simulink model "soft_robot_model"  (R2025b)
settings: Solver=VariableStepAuto  StartTime=0.0  StopTime=10.0  RelTol=1e-3
values from neighbouring files (symbols this model uses):
  d_z = 0    [Code4Simulink.m]
  L = 0.15    [Code4Simulink.m]
  phi = [30, 150, 270] * pi/180    [Code4Simulink.m]
  theta_x = deg2rad(0)    [Code4Simulink.m]
  theta_y = deg2rad(0)    [Code4Simulink.m]
undefined symbols (not defined in the file or in its folder): X, Y, Z
libraries: sm_lib x23, nesl_utility x4
settings Model: Creator=didar  LastModifiedBy=didar

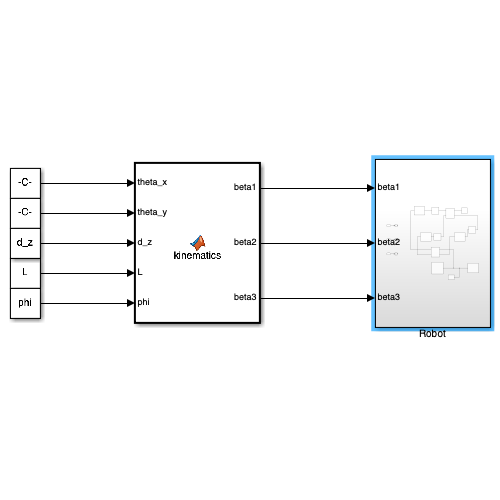
[thumbnail: Simulink's stored preview of the top-level diagram]
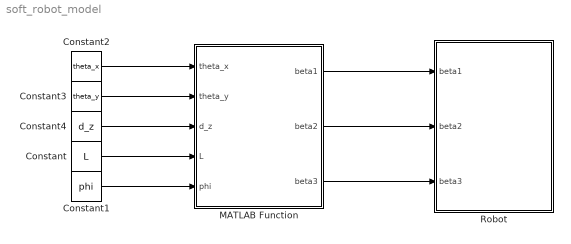
== system soft_robot_model ==
  Constant : Constant  Value=L
  Constant1 : Constant  Value=phi
  Constant2 : Constant  Value=theta_x
  Constant3 : Constant  Value=theta_y
  Constant4 : Constant  Value=d_z
  MATLAB Function : MATLAB Function  TreatAsAtomicUnit=on
  Robot : Subsystem
  wires:
  Constant1/1 -> MATLAB Function/5(phi)
  Constant/1 -> MATLAB Function/4(L)
  Constant2/1 -> MATLAB Function/1(theta_x)
  Constant3/1 -> MATLAB Function/2(theta_y)
  Constant4/1 -> MATLAB Function/3(d_z)
  MATLAB Function/1(beta1) -> Robot/1(beta1)
  MATLAB Function/2(beta2) -> Robot/2(beta2)
  MATLAB Function/3(beta3) -> Robot/3(beta3)

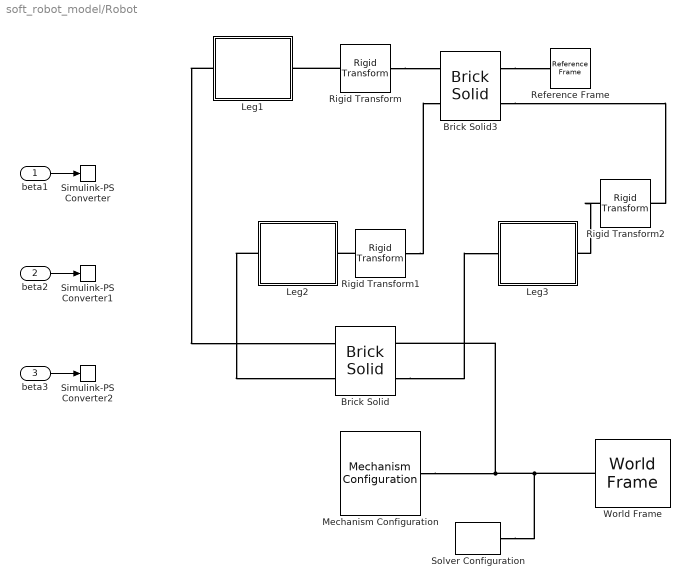
== system soft_robot_model/Robot ==
  beta1 : Inport
  beta2 : Inport  Port=2
  beta3 : Inport  Port=3
  Brick Solid : sm_lib/Body Elements/Brick Solid  BrickDimensions=[10 10 1]  BrickDimensionsUnits=cm  ExportEntireGeometry=off  InertiaType=CalculateFromGeometry  BasedOnType=Density  Density=1000  DensityUnits=kg/m^3  Mass=1  MassUnits=kg  CenterOfMass=[0 0 0]  CenterOfMassUnits=m  MomentsOfInertia=[1 1 1]  MomentsOfInertiaUnits=kg*m^2  ProductsOfInertia=[0 0 0]  ProductsOfInertiaUnits=kg*m^2  GraphicType=FromGeometry  MarkerShape=Sphere  MarkerSize=10  GraphicVisPropType=SimpleVisualProperties  GraphicDiffuseColor=[0.5 0.5 0.5]  GraphicOpacity=1  GraphicSpecularColor=[0.5 0.5 0.5 1.0]  GraphicAmbientColor=[0.15 0.15 0.15 1.0]  GraphicEmissiveColor=[0.0 0.0 0.0 1.0]  GraphicShininess=75  DoExposeReferenceFrame=on  SerializedFrames=<Frames><Frame><Id>Frame1</Id><Value><Name>F1</Name><Origin><Source>ReferenceFrame</Source><FeatureName></FeatureName></Origin><PrimaryAxis><DefinedDirection>+Z</DefinedDirection><Source>ReferenceFrame</Source><SourceDirection>+Z</SourceDirection><FeatureName></FeatureName></PrimaryAxis><SecondaryAxis><DefinedDirection>+X</DefinedDirection><Source>ReferenceFrame</Source><SourceDirection>+X</SourceDirection><FeatureName></FeatureName></SecondaryAxis></Value></Frame><Frame><Id>Frame2</Id><Value><Name>F2</Name><Origin><Source>ReferenceFrame</Source><FeatureName></FeatureName></Origin><PrimaryAxis><DefinedDirection>+Z</DefinedDirection><Source>ReferenceFrame</Source><SourceDirection>+Z</SourceDirection><FeatureName></FeatureName></PrimaryAxis><SecondaryAxis><DefinedDirection>+X</DefinedDirection><Source>ReferenceFrame</Source><SourceDirection>+X</SourceDirection><FeatureName></FeatureName></SecondaryAxis></Value></Frame><Frame><Id>Frame3</Id><Value><Name>F3</Name><Origin><Source>ReferenceFrame</Source><FeatureName></FeatureName></Origin><PrimaryAxis><DefinedDirection>+Z</DefinedDirection><Source>ReferenceFrame</Source><SourceDirection>+Z</SourceDirection><FeatureName></FeatureName></PrimaryAxis><SecondaryAxis><DefinedDirection>+X</DefinedDirection><Source>ReferenceFrame</Source><SourceDirection>+X</SourceDirection><FeatureName></FeatureName></SecondaryAxis></Value></Frame></Frames>
  Brick Solid3 : sm_lib/Body Elements/Brick Solid  BrickDimensions=[10 10 1]  BrickDimensionsUnits=cm  ExportEntireGeometry=off  InertiaType=CalculateFromGeometry  BasedOnType=Density  Density=1000  DensityUnits=kg/m^3  Mass=1  MassUnits=kg  CenterOfMass=[0 0 0]  CenterOfMassUnits=m  MomentsOfInertia=[1 1 1]  MomentsOfInertiaUnits=kg*m^2  ProductsOfInertia=[0 0 0]  ProductsOfInertiaUnits=kg*m^2  GraphicType=FromGeometry  MarkerShape=Sphere  MarkerSize=10  GraphicVisPropType=SimpleVisualProperties  GraphicDiffuseColor=[0.5 0.5 0.5]  GraphicOpacity=1  GraphicSpecularColor=[0.5 0.5 0.5 1.0]  GraphicAmbientColor=[0.15 0.15 0.15 1.0]  GraphicEmissiveColor=[0.0 0.0 0.0 1.0]  GraphicShininess=75  DoExposeReferenceFrame=on  SerializedFrames=<Frames><Frame><Id>Frame1</Id><Value><Name>F1</Name><Origin><Source>ReferenceFrame</Source><FeatureName></FeatureName></Origin><PrimaryAxis><DefinedDirection>+Z</DefinedDirection><Source>ReferenceFrame</Source><SourceDirection>+Z</SourceDirection><FeatureName></FeatureName></PrimaryAxis><SecondaryAxis><DefinedDirection>+X</DefinedDirection><Source>ReferenceFrame</Source><SourceDirection>+X</SourceDirection><FeatureName></FeatureName></SecondaryAxis></Value></Frame><Frame><Id>Frame2</Id><Value><Name>F2</Name><Origin><Source>ReferenceFrame</Source><FeatureName></FeatureName></Origin><PrimaryAxis><DefinedDirection>+Z</DefinedDirection><Source>ReferenceFrame</Source><SourceDirection>+Z</SourceDirection><FeatureName></FeatureName></PrimaryAxis><SecondaryAxis><DefinedDirection>+X</DefinedDirection><Source>ReferenceFrame</Source><SourceDirection>+X</SourceDirection><FeatureName></FeatureName></SecondaryAxis></Value></Frame><Frame><Id>Frame3</Id><Value><Name>F3</Name><Origin><Source>ReferenceFrame</Source><FeatureName></FeatureName></Origin><PrimaryAxis><DefinedDirection>+Z</DefinedDirection><Source>ReferenceFrame</Source><SourceDirection>+Z</SourceDirection><FeatureName></FeatureName></PrimaryAxis><SecondaryAxis><DefinedDirection>+X</DefinedDirection><Source>ReferenceFrame</Source><SourceDirection>+X</SourceDirection><FeatureName></FeatureName></SecondaryAxis></Value></Frame></Frames>
  Leg1 : Subsystem
  Leg2 : Subsystem
  Leg3 : Subsystem
  Mechanism Configuration : sm_lib/Utilities/Mechanism Configuration  UniformGravity=Constant  GravityVector=[0 0 -9.80665]  GravityVectorUnits=m/s^2  LinearizationDelta=0.001  JointModeTransitionNonlinearIterations=2
  Reference Frame : sm_lib/Frames and Transforms/Reference Frame
  Rigid Transform : sm_lib/Frames and Transforms/Rigid Transform  RotationMethod=StandardAxis  FollAlignAxisA=+X  BaseAlignAxisA=+Y  FollAlignAxisB=+Y  BaseAlignAxisB=+Z  RotationStandardAxis=+Z  RotationAngle=30  RotationAngleUnits=deg  RotationArbitraryAxis=[0 0 1]  RotationSequenceAxes=FollowerAxes  RotationSequence=XYX  RotationSequenceAngles=[0 0 0]  RotationSequenceAnglesUnits=deg  RotationMatrix=[1 0 0;0 1 0;0 0 1]  Quaternion=[1 0 0 0]  TranslationMethod=None  TranslationCartesianOffset=[0 0 0]  TranslationCartesianOffsetUnits=m  TranslationStandardAxis=+Z  TranslationStandardOffset=0  TranslationStandardOffsetUnits=m  TranslationROffset=0  TranslationROffsetUnits=m  TranslationThetaOffset=0  TranslationThetaOffsetUnits=deg  TranslationZOffset=0  TranslationZOffsetUnits=m
  Rigid Transform1 : sm_lib/Frames and Transforms/Rigid Transform  RotationMethod=StandardAxis  FollAlignAxisA=+X  BaseAlignAxisA=+Y  FollAlignAxisB=+Y  BaseAlignAxisB=+Z  RotationStandardAxis=+Z  RotationAngle=150  RotationAngleUnits=deg  RotationArbitraryAxis=[0 0 1]  RotationSequenceAxes=FollowerAxes  RotationSequence=XYX  RotationSequenceAngles=[0 0 0]  RotationSequenceAnglesUnits=deg  RotationMatrix=[1 0 0;0 1 0;0 0 1]  Quaternion=[1 0 0 0]  TranslationMethod=None  TranslationCartesianOffset=[0 0 0]  TranslationCartesianOffsetUnits=m  TranslationStandardAxis=+Z  TranslationStandardOffset=0  TranslationStandardOffsetUnits=m  TranslationROffset=0  TranslationROffsetUnits=m  TranslationThetaOffset=0  TranslationThetaOffsetUnits=deg  TranslationZOffset=0  TranslationZOffsetUnits=m
  Rigid Transform2 : sm_lib/Frames and Transforms/Rigid Transform  RotationMethod=StandardAxis  FollAlignAxisA=+X  BaseAlignAxisA=+Y  FollAlignAxisB=+Y  BaseAlignAxisB=+Z  RotationStandardAxis=+Z  RotationAngle=270  RotationAngleUnits=deg  RotationArbitraryAxis=[0 0 1]  RotationSequenceAxes=FollowerAxes  RotationSequence=XYX  RotationSequenceAngles=[0 0 0]  RotationSequenceAnglesUnits=deg  RotationMatrix=[1 0 0;0 1 0;0 0 1]  Quaternion=[1 0 0 0]  TranslationMethod=None  TranslationCartesianOffset=[0 0 0]  TranslationCartesianOffsetUnits=m  TranslationStandardAxis=+Z  TranslationStandardOffset=0  TranslationStandardOffsetUnits=m  TranslationROffset=0  TranslationROffsetUnits=m  TranslationThetaOffset=0  TranslationThetaOffsetUnits=deg  TranslationZOffset=0  TranslationZOffsetUnits=m
  Simulink-PS Converter : nesl_utility/Simulink-PS Converter  PhysicalDomain=network_engine_domain  SubClassName=ps_input  LeftPortType=input  RightPortType=output  PseudoPeriodic=off  Frequencies=[]  NoiseDistribution=none  NoiseParameters=[]  Unit=1  AffineConversion=off  FilteringAndDerivatives=provide  SimscapeFilterOrder=1  InputFilterTimeConstant=0.001  UdotUserProvided=0
  Simulink-PS Converter1 : nesl_utility/Simulink-PS Converter  PhysicalDomain=network_engine_domain  SubClassName=ps_input  LeftPortType=input  RightPortType=output  PseudoPeriodic=off  Frequencies=[]  NoiseDistribution=none  NoiseParameters=[]  Unit=1  AffineConversion=off  FilteringAndDerivatives=provide  SimscapeFilterOrder=1  InputFilterTimeConstant=0.001  UdotUserProvided=0
  Simulink-PS Converter2 : nesl_utility/Simulink-PS Converter  PhysicalDomain=network_engine_domain  SubClassName=ps_input  LeftPortType=input  RightPortType=output  PseudoPeriodic=off  Frequencies=[]  NoiseDistribution=none  NoiseParameters=[]  Unit=1  AffineConversion=off  FilteringAndDerivatives=provide  SimscapeFilterOrder=1  InputFilterTimeConstant=0.001  UdotUserProvided=0
  Solver Configuration : nesl_utility/Solver Configuration  PhysicalDomain=network_engine_domain  SubClassName=solver  LeftPortType=input  RightPortType=generic  Tones=[]  Harmonics=[]  SimulateNoise=off  Profile=off  UseLocalSampling=off  EnableSwitchedLinearOptims=on  FrequencyDomain=off  UseCCode=off  RelTol=0.001  AbsTol=0.001  MinStep=1e-09  ToWorkspace=off  RevertToSquareIcSolve=off  NumHomotopyIterations=100  PhasorMode=off  PhasorModeNumHarmonics=1  ConsistencySolver=NEWTON_XTOL_AFTER_FTOL  IndexReductionMethod=DerivativeReplacement  DoDC=off  ResidualTolerance=1e-09  ConsistencyTolSource=GLOBAL  ConsistencyAbsTol=0.001  ConsistencyRelTol=0.001  ConsistencyTolFactor=0.001  UseLocalSolver=off  LocalSolverChoice=NE_BACKWARD_EULER_ADVANCER  ResolveIndetEquations=on  FunctionEvalNumThread=1  LocalSolverSampleTime=0.001  DoFixedCost=off  MaxNonlinIter=3  MaxModeIter=2  ComputeImpulses=off  ImpulseIterations=2  LinearAlgebra=auto  LinearAlgebraNumThread=0  EquationFormulation=NE_TIME_EF  DelaysMemoryBudget=1024  AutomaticFiltering=on  FilteringTimeConstant=0.001  PartitionStorageMethod=AS_NEEDED  PartitionMemoryBudget=1024  PartitionMethod=ROBUST  MultibodyUseLocalSolver=off  MultibodyLocalSolverChoice=ODE1  MultibodyLocalSolverSampleTime=0.001
  World Frame : sm_lib/Frames and Transforms/World Frame
  wires:
  beta1/1 -> Simulink-PS Converter/1
  beta2/1 -> Simulink-PS Converter1/1
  beta3/1 -> Simulink-PS Converter2/1
  connections:
  World Frame/RConn1 -- Solver Configuration/RConn1 -- Brick Solid/RConn1 -- Mechanism Configuration/RConn1
  Leg1/RConn1 -- Brick Solid/LConn1
  Leg2/RConn1 -- Brick Solid/LConn2
  Brick Solid/RConn2 -- Leg3/RConn1
  Rigid Transform/LConn1 -- Leg1/LConn1
  Rigid Transform/RConn1 -- Brick Solid3/LConn1
  Rigid Transform1/LConn1 -- Leg2/LConn1
  Rigid Transform1/RConn1 -- Brick Solid3/LConn2
  Rigid Transform2/LConn1 -- Leg3/LConn1
  Brick Solid3/RConn2 -- Rigid Transform2/RConn1
  Brick Solid3/RConn1 -- Reference Frame/RConn1

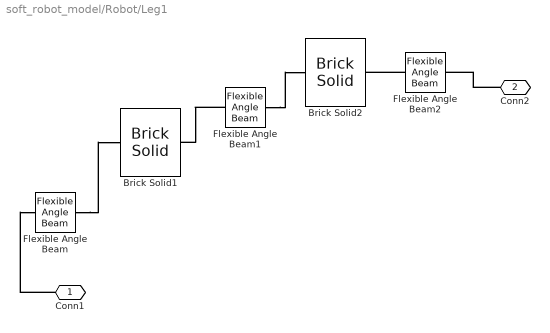
== system soft_robot_model/Robot/Leg1 ==
  Brick Solid1 : sm_lib/Body Elements/Brick Solid  BrickDimensions=[4.5 0.7 8.6]  BrickDimensionsUnits=cm  ExportEntireGeometry=off  InertiaType=CalculateFromGeometry  BasedOnType=Density  Density=1000  DensityUnits=kg/m^3  Mass=1  MassUnits=kg  CenterOfMass=[0 0 0]  CenterOfMassUnits=m  MomentsOfInertia=[1 1 1]  MomentsOfInertiaUnits=kg*m^2  ProductsOfInertia=[0 0 0]  ProductsOfInertiaUnits=kg*m^2  GraphicType=FromGeometry  MarkerShape=Sphere  MarkerSize=10  GraphicVisPropType=SimpleVisualProperties  GraphicDiffuseColor=[0.5 0.5 0.5]  GraphicOpacity=1  GraphicSpecularColor=[0.5 0.5 0.5 1.0]  GraphicAmbientColor=[0.15 0.15 0.15 1.0]  GraphicEmissiveColor=[0.0 0.0 0.0 1.0]  GraphicShininess=75  DoExposeReferenceFrame=on  SerializedFrames=<Frames><Frame><Id>Frame1</Id><Value><Name>F1</Name><Origin><Source>ReferenceFrame</Source><FeatureName></FeatureName></Origin><PrimaryAxis><DefinedDirection>+Z</DefinedDirection><Source>ReferenceFrame</Source><SourceDirection>+Z</SourceDirection><FeatureName></FeatureName></PrimaryAxis><SecondaryAxis><DefinedDirection>+X</DefinedDirection><Source>ReferenceFrame</Source><SourceDirection>+X</SourceDirection><FeatureName></FeatureName></SecondaryAxis></Value></Frame></Frames>
  Brick Solid2 : sm_lib/Body Elements/Brick Solid  BrickDimensions=[4.5 0.7 8.6]  BrickDimensionsUnits=cm  ExportEntireGeometry=off  InertiaType=CalculateFromGeometry  BasedOnType=Density  Density=1000  DensityUnits=kg/m^3  Mass=1  MassUnits=kg  CenterOfMass=[0 0 0]  CenterOfMassUnits=m  MomentsOfInertia=[1 1 1]  MomentsOfInertiaUnits=kg*m^2  ProductsOfInertia=[0 0 0]  ProductsOfInertiaUnits=kg*m^2  GraphicType=FromGeometry  MarkerShape=Sphere  MarkerSize=10  GraphicVisPropType=SimpleVisualProperties  GraphicDiffuseColor=[0.5 0.5 0.5]  GraphicOpacity=1  GraphicSpecularColor=[0.5 0.5 0.5 1.0]  GraphicAmbientColor=[0.15 0.15 0.15 1.0]  GraphicEmissiveColor=[0.0 0.0 0.0 1.0]  GraphicShininess=75  DoExposeReferenceFrame=on  SerializedFrames=<Frames><Frame><Id>Frame1</Id><Value><Name>F1</Name><Origin><Source>ReferenceFrame</Source><FeatureName></FeatureName></Origin><PrimaryAxis><DefinedDirection>+Z</DefinedDirection><Source>ReferenceFrame</Source><SourceDirection>+Z</SourceDirection><FeatureName></FeatureName></PrimaryAxis><SecondaryAxis><DefinedDirection>+X</DefinedDirection><Source>ReferenceFrame</Source><SourceDirection>+X</SourceDirection><FeatureName></FeatureName></SecondaryAxis></Value></Frame></Frames>
  Flexible Angle Beam : sm_lib/Body Elements/Flexible Bodies/Beams/Flexible Angle Beam  EndToEndWidth=1  EndToEndWidthUnits=m  EndToEndHeight=1  EndToEndHeightUnits=m  VerticalLegThickness=0.1  VerticalLegThicknessUnits=m  HorizontalLegThickness=0.1  HorizontalLegThicknessUnits=m  Length=10  LengthUnits=m  StiffnessAndInertiaType=CalculateFromGeometry  Density=2700  DensityUnits=kg/m^3  ModuliType=YoungsPoissons  YoungsModulus=70  YoungsModulusUnits=GPa  PoissonsRatio=0.33  ShearModulus=26  ShearModulusUnits=GPa  GeometricCentroid=[0 0]  GeometricCentroidUnits=m  BendingCentroid=[0 0]  BendingCentroidUnits=m  ShearCenter=[0 0]  ShearCenterUnits=m  AxialRigidity=1  AxialRigidityUnits=Pa*m^2  FlexuralRigidity=[1 1]  FlexuralRigidityUnits=Pa*m^4  CrossFlexuralRigidity=0  CrossFlexuralRigidityUnits=Pa*m^4  TorsionalRigidity=1  TorsionalRigidityUnits=Pa*m^4  CenterOfMass=[0 0]  CenterOfMassUnits=m  MassPerUnitLength=1  MassPerUnitLengthUnits=kg/m  MassMomentOfInertiaDensity=[1 1]  MassMomentOfInertiaDensityUnits=kg*m  MassProductOfInertiaDensity=0  MassProductOfInertiaDensityUnits=kg*m  DampingType=Proportional  ProportionalDampingAlpha=0  ProportionalDampingAlphaUnits=1/s  ProportionalDampingBeta=0.001  ProportionalDampingBetaUnits=s  UniformModalDampingRatio=0.01  NumElements=1  ReferenceConditionsType=LinearizedMeanAxes  DoExposeReferenceFrame=off  ReductionType=None  NumRetainedModes=1  GraphicType=FromGeometry  GraphicVisPropType=SimpleVisualProperties  GraphicDiffuseColor=[0.5 0.5 0.5]  GraphicOpacity=1  GraphicSpecularColor=[0.5 0.5 0.5 1.0]  GraphicAmbientColor=[0.15 0.15 0.15 1.0]  GraphicEmissiveColor=[0.0 0.0 0.0 1.0]  GraphicShininess=75  DoExposeZminFrame=on  DoExposeZmaxFrame=on  SerializedFrames=<Frames/>
  Flexible Angle Beam1 : sm_lib/Body Elements/Flexible Bodies/Beams/Flexible Angle Beam  EndToEndWidth=1  EndToEndWidthUnits=m  EndToEndHeight=1  EndToEndHeightUnits=m  VerticalLegThickness=0.1  VerticalLegThicknessUnits=m  HorizontalLegThickness=0.1  HorizontalLegThicknessUnits=m  Length=10  LengthUnits=m  StiffnessAndInertiaType=CalculateFromGeometry  Density=2700  DensityUnits=kg/m^3  ModuliType=YoungsPoissons  YoungsModulus=70  YoungsModulusUnits=GPa  PoissonsRatio=0.33  ShearModulus=26  ShearModulusUnits=GPa  GeometricCentroid=[0 0]  GeometricCentroidUnits=m  BendingCentroid=[0 0]  BendingCentroidUnits=m  ShearCenter=[0 0]  ShearCenterUnits=m  AxialRigidity=1  AxialRigidityUnits=Pa*m^2  FlexuralRigidity=[1 1]  FlexuralRigidityUnits=Pa*m^4  CrossFlexuralRigidity=0  CrossFlexuralRigidityUnits=Pa*m^4  TorsionalRigidity=1  TorsionalRigidityUnits=Pa*m^4  CenterOfMass=[0 0]  CenterOfMassUnits=m  MassPerUnitLength=1  MassPerUnitLengthUnits=kg/m  MassMomentOfInertiaDensity=[1 1]  MassMomentOfInertiaDensityUnits=kg*m  MassProductOfInertiaDensity=0  MassProductOfInertiaDensityUnits=kg*m  DampingType=Proportional  ProportionalDampingAlpha=0  ProportionalDampingAlphaUnits=1/s  ProportionalDampingBeta=0.001  ProportionalDampingBetaUnits=s  UniformModalDampingRatio=0.01  NumElements=1  ReferenceConditionsType=LinearizedMeanAxes  DoExposeReferenceFrame=off  ReductionType=None  NumRetainedModes=1  GraphicType=FromGeometry  GraphicVisPropType=SimpleVisualProperties  GraphicDiffuseColor=[0.5 0.5 0.5]  GraphicOpacity=1  GraphicSpecularColor=[0.5 0.5 0.5 1.0]  GraphicAmbientColor=[0.15 0.15 0.15 1.0]  GraphicEmissiveColor=[0.0 0.0 0.0 1.0]  GraphicShininess=75  DoExposeZminFrame=on  DoExposeZmaxFrame=on  SerializedFrames=<Frames/>
  Flexible Angle Beam2 : sm_lib/Body Elements/Flexible Bodies/Beams/Flexible Angle Beam  EndToEndWidth=1  EndToEndWidthUnits=m  EndToEndHeight=1  EndToEndHeightUnits=m  VerticalLegThickness=0.1  VerticalLegThicknessUnits=m  HorizontalLegThickness=0.1  HorizontalLegThicknessUnits=m  Length=10  LengthUnits=m  StiffnessAndInertiaType=CalculateFromGeometry  Density=2700  DensityUnits=kg/m^3  ModuliType=YoungsPoissons  YoungsModulus=70  YoungsModulusUnits=GPa  PoissonsRatio=0.33  ShearModulus=26  ShearModulusUnits=GPa  GeometricCentroid=[0 0]  GeometricCentroidUnits=m  BendingCentroid=[0 0]  BendingCentroidUnits=m  ShearCenter=[0 0]  ShearCenterUnits=m  AxialRigidity=1  AxialRigidityUnits=Pa*m^2  FlexuralRigidity=[1 1]  FlexuralRigidityUnits=Pa*m^4  CrossFlexuralRigidity=0  CrossFlexuralRigidityUnits=Pa*m^4  TorsionalRigidity=1  TorsionalRigidityUnits=Pa*m^4  CenterOfMass=[0 0]  CenterOfMassUnits=m  MassPerUnitLength=1  MassPerUnitLengthUnits=kg/m  MassMomentOfInertiaDensity=[1 1]  MassMomentOfInertiaDensityUnits=kg*m  MassProductOfInertiaDensity=0  MassProductOfInertiaDensityUnits=kg*m  DampingType=Proportional  ProportionalDampingAlpha=0  ProportionalDampingAlphaUnits=1/s  ProportionalDampingBeta=0.001  ProportionalDampingBetaUnits=s  UniformModalDampingRatio=0.01  NumElements=1  ReferenceConditionsType=LinearizedMeanAxes  DoExposeReferenceFrame=off  ReductionType=None  NumRetainedModes=1  GraphicType=FromGeometry  GraphicVisPropType=SimpleVisualProperties  GraphicDiffuseColor=[0.5 0.5 0.5]  GraphicOpacity=1  GraphicSpecularColor=[0.5 0.5 0.5 1.0]  GraphicAmbientColor=[0.15 0.15 0.15 1.0]  GraphicEmissiveColor=[0.0 0.0 0.0 1.0]  GraphicShininess=75  DoExposeZminFrame=on  DoExposeZmaxFrame=on  SerializedFrames=<Frames/>
  Conn1 : PMIOPort  Side=Right
  Conn2 : PMIOPort  Port=2  Side=Left
  connections:
  Flexible Angle Beam/RConn1 -- Brick Solid1/LConn1
  Flexible Angle Beam2/LConn1 -- Brick Solid2/RConn1
  Flexible Angle Beam1/LConn1 -- Brick Solid1/RConn1
  Conn1/RConn1 -- Flexible Angle Beam/LConn1
  Flexible Angle Beam1/RConn1 -- Brick Solid2/LConn1
  Conn2/RConn1 -- Flexible Angle Beam2/RConn1

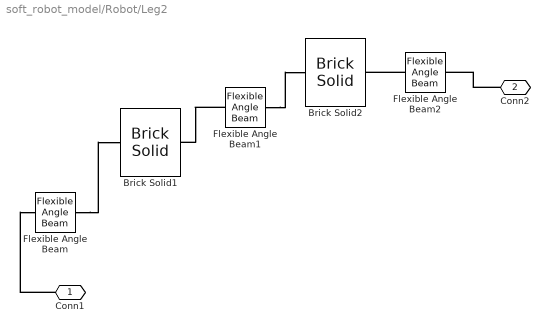
== system soft_robot_model/Robot/Leg2 ==
  Brick Solid1 : sm_lib/Body Elements/Brick Solid  BrickDimensions=[4.5 0.7 8.6]  BrickDimensionsUnits=cm  ExportEntireGeometry=off  InertiaType=CalculateFromGeometry  BasedOnType=Density  Density=1000  DensityUnits=kg/m^3  Mass=1  MassUnits=kg  CenterOfMass=[0 0 0]  CenterOfMassUnits=m  MomentsOfInertia=[1 1 1]  MomentsOfInertiaUnits=kg*m^2  ProductsOfInertia=[0 0 0]  ProductsOfInertiaUnits=kg*m^2  GraphicType=FromGeometry  MarkerShape=Sphere  MarkerSize=10  GraphicVisPropType=SimpleVisualProperties  GraphicDiffuseColor=[0.5 0.5 0.5]  GraphicOpacity=1  GraphicSpecularColor=[0.5 0.5 0.5 1.0]  GraphicAmbientColor=[0.15 0.15 0.15 1.0]  GraphicEmissiveColor=[0.0 0.0 0.0 1.0]  GraphicShininess=75  DoExposeReferenceFrame=on  SerializedFrames=<Frames><Frame><Id>Frame1</Id><Value><Name>F1</Name><Origin><Source>ReferenceFrame</Source><FeatureName></FeatureName></Origin><PrimaryAxis><DefinedDirection>+Z</DefinedDirection><Source>ReferenceFrame</Source><SourceDirection>+Z</SourceDirection><FeatureName></FeatureName></PrimaryAxis><SecondaryAxis><DefinedDirection>+X</DefinedDirection><Source>ReferenceFrame</Source><SourceDirection>+X</SourceDirection><FeatureName></FeatureName></SecondaryAxis></Value></Frame></Frames>
  Brick Solid2 : sm_lib/Body Elements/Brick Solid  BrickDimensions=[4.5 0.7 8.6]  BrickDimensionsUnits=cm  ExportEntireGeometry=off  InertiaType=CalculateFromGeometry  BasedOnType=Density  Density=1000  DensityUnits=kg/m^3  Mass=1  MassUnits=kg  CenterOfMass=[0 0 0]  CenterOfMassUnits=m  MomentsOfInertia=[1 1 1]  MomentsOfInertiaUnits=kg*m^2  ProductsOfInertia=[0 0 0]  ProductsOfInertiaUnits=kg*m^2  GraphicType=FromGeometry  MarkerShape=Sphere  MarkerSize=10  GraphicVisPropType=SimpleVisualProperties  GraphicDiffuseColor=[0.5 0.5 0.5]  GraphicOpacity=1  GraphicSpecularColor=[0.5 0.5 0.5 1.0]  GraphicAmbientColor=[0.15 0.15 0.15 1.0]  GraphicEmissiveColor=[0.0 0.0 0.0 1.0]  GraphicShininess=75  DoExposeReferenceFrame=on  SerializedFrames=<Frames><Frame><Id>Frame1</Id><Value><Name>F1</Name><Origin><Source>ReferenceFrame</Source><FeatureName></FeatureName></Origin><PrimaryAxis><DefinedDirection>+Z</DefinedDirection><Source>ReferenceFrame</Source><SourceDirection>+Z</SourceDirection><FeatureName></FeatureName></PrimaryAxis><SecondaryAxis><DefinedDirection>+X</DefinedDirection><Source>ReferenceFrame</Source><SourceDirection>+X</SourceDirection><FeatureName></FeatureName></SecondaryAxis></Value></Frame></Frames>
  Flexible Angle Beam : sm_lib/Body Elements/Flexible Bodies/Beams/Flexible Angle Beam  EndToEndWidth=1  EndToEndWidthUnits=m  EndToEndHeight=1  EndToEndHeightUnits=m  VerticalLegThickness=0.1  VerticalLegThicknessUnits=m  HorizontalLegThickness=0.1  HorizontalLegThicknessUnits=m  Length=10  LengthUnits=m  StiffnessAndInertiaType=CalculateFromGeometry  Density=2700  DensityUnits=kg/m^3  ModuliType=YoungsPoissons  YoungsModulus=70  YoungsModulusUnits=GPa  PoissonsRatio=0.33  ShearModulus=26  ShearModulusUnits=GPa  GeometricCentroid=[0 0]  GeometricCentroidUnits=m  BendingCentroid=[0 0]  BendingCentroidUnits=m  ShearCenter=[0 0]  ShearCenterUnits=m  AxialRigidity=1  AxialRigidityUnits=Pa*m^2  FlexuralRigidity=[1 1]  FlexuralRigidityUnits=Pa*m^4  CrossFlexuralRigidity=0  CrossFlexuralRigidityUnits=Pa*m^4  TorsionalRigidity=1  TorsionalRigidityUnits=Pa*m^4  CenterOfMass=[0 0]  CenterOfMassUnits=m  MassPerUnitLength=1  MassPerUnitLengthUnits=kg/m  MassMomentOfInertiaDensity=[1 1]  MassMomentOfInertiaDensityUnits=kg*m  MassProductOfInertiaDensity=0  MassProductOfInertiaDensityUnits=kg*m  DampingType=Proportional  ProportionalDampingAlpha=0  ProportionalDampingAlphaUnits=1/s  ProportionalDampingBeta=0.001  ProportionalDampingBetaUnits=s  UniformModalDampingRatio=0.01  NumElements=1  ReferenceConditionsType=LinearizedMeanAxes  DoExposeReferenceFrame=off  ReductionType=None  NumRetainedModes=1  GraphicType=FromGeometry  GraphicVisPropType=SimpleVisualProperties  GraphicDiffuseColor=[0.5 0.5 0.5]  GraphicOpacity=1  GraphicSpecularColor=[0.5 0.5 0.5 1.0]  GraphicAmbientColor=[0.15 0.15 0.15 1.0]  GraphicEmissiveColor=[0.0 0.0 0.0 1.0]  GraphicShininess=75  DoExposeZminFrame=on  DoExposeZmaxFrame=on  SerializedFrames=<Frames/>
  Flexible Angle Beam1 : sm_lib/Body Elements/Flexible Bodies/Beams/Flexible Angle Beam  EndToEndWidth=1  EndToEndWidthUnits=m  EndToEndHeight=1  EndToEndHeightUnits=m  VerticalLegThickness=0.1  VerticalLegThicknessUnits=m  HorizontalLegThickness=0.1  HorizontalLegThicknessUnits=m  Length=10  LengthUnits=m  StiffnessAndInertiaType=CalculateFromGeometry  Density=2700  DensityUnits=kg/m^3  ModuliType=YoungsPoissons  YoungsModulus=70  YoungsModulusUnits=GPa  PoissonsRatio=0.33  ShearModulus=26  ShearModulusUnits=GPa  GeometricCentroid=[0 0]  GeometricCentroidUnits=m  BendingCentroid=[0 0]  BendingCentroidUnits=m  ShearCenter=[0 0]  ShearCenterUnits=m  AxialRigidity=1  AxialRigidityUnits=Pa*m^2  FlexuralRigidity=[1 1]  FlexuralRigidityUnits=Pa*m^4  CrossFlexuralRigidity=0  CrossFlexuralRigidityUnits=Pa*m^4  TorsionalRigidity=1  TorsionalRigidityUnits=Pa*m^4  CenterOfMass=[0 0]  CenterOfMassUnits=m  MassPerUnitLength=1  MassPerUnitLengthUnits=kg/m  MassMomentOfInertiaDensity=[1 1]  MassMomentOfInertiaDensityUnits=kg*m  MassProductOfInertiaDensity=0  MassProductOfInertiaDensityUnits=kg*m  DampingType=Proportional  ProportionalDampingAlpha=0  ProportionalDampingAlphaUnits=1/s  ProportionalDampingBeta=0.001  ProportionalDampingBetaUnits=s  UniformModalDampingRatio=0.01  NumElements=1  ReferenceConditionsType=LinearizedMeanAxes  DoExposeReferenceFrame=off  ReductionType=None  NumRetainedModes=1  GraphicType=FromGeometry  GraphicVisPropType=SimpleVisualProperties  GraphicDiffuseColor=[0.5 0.5 0.5]  GraphicOpacity=1  GraphicSpecularColor=[0.5 0.5 0.5 1.0]  GraphicAmbientColor=[0.15 0.15 0.15 1.0]  GraphicEmissiveColor=[0.0 0.0 0.0 1.0]  GraphicShininess=75  DoExposeZminFrame=on  DoExposeZmaxFrame=on  SerializedFrames=<Frames/>
  Flexible Angle Beam2 : sm_lib/Body Elements/Flexible Bodies/Beams/Flexible Angle Beam  EndToEndWidth=1  EndToEndWidthUnits=m  EndToEndHeight=1  EndToEndHeightUnits=m  VerticalLegThickness=0.1  VerticalLegThicknessUnits=m  HorizontalLegThickness=0.1  HorizontalLegThicknessUnits=m  Length=10  LengthUnits=m  StiffnessAndInertiaType=CalculateFromGeometry  Density=2700  DensityUnits=kg/m^3  ModuliType=YoungsPoissons  YoungsModulus=70  YoungsModulusUnits=GPa  PoissonsRatio=0.33  ShearModulus=26  ShearModulusUnits=GPa  GeometricCentroid=[0 0]  GeometricCentroidUnits=m  BendingCentroid=[0 0]  BendingCentroidUnits=m  ShearCenter=[0 0]  ShearCenterUnits=m  AxialRigidity=1  AxialRigidityUnits=Pa*m^2  FlexuralRigidity=[1 1]  FlexuralRigidityUnits=Pa*m^4  CrossFlexuralRigidity=0  CrossFlexuralRigidityUnits=Pa*m^4  TorsionalRigidity=1  TorsionalRigidityUnits=Pa*m^4  CenterOfMass=[0 0]  CenterOfMassUnits=m  MassPerUnitLength=1  MassPerUnitLengthUnits=kg/m  MassMomentOfInertiaDensity=[1 1]  MassMomentOfInertiaDensityUnits=kg*m  MassProductOfInertiaDensity=0  MassProductOfInertiaDensityUnits=kg*m  DampingType=Proportional  ProportionalDampingAlpha=0  ProportionalDampingAlphaUnits=1/s  ProportionalDampingBeta=0.001  ProportionalDampingBetaUnits=s  UniformModalDampingRatio=0.01  NumElements=1  ReferenceConditionsType=LinearizedMeanAxes  DoExposeReferenceFrame=off  ReductionType=None  NumRetainedModes=1  GraphicType=FromGeometry  GraphicVisPropType=SimpleVisualProperties  GraphicDiffuseColor=[0.5 0.5 0.5]  GraphicOpacity=1  GraphicSpecularColor=[0.5 0.5 0.5 1.0]  GraphicAmbientColor=[0.15 0.15 0.15 1.0]  GraphicEmissiveColor=[0.0 0.0 0.0 1.0]  GraphicShininess=75  DoExposeZminFrame=on  DoExposeZmaxFrame=on  SerializedFrames=<Frames/>
  Conn1 : PMIOPort  Side=Right
  Conn2 : PMIOPort  Port=2  Side=Left
  connections:
  Flexible Angle Beam/RConn1 -- Brick Solid1/LConn1
  Flexible Angle Beam2/LConn1 -- Brick Solid2/RConn1
  Flexible Angle Beam1/LConn1 -- Brick Solid1/RConn1
  Conn1/RConn1 -- Flexible Angle Beam/LConn1
  Flexible Angle Beam1/RConn1 -- Brick Solid2/LConn1
  Conn2/RConn1 -- Flexible Angle Beam2/RConn1

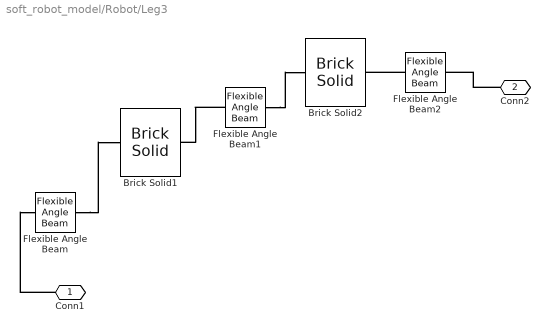
== system soft_robot_model/Robot/Leg3 ==
  Brick Solid1 : sm_lib/Body Elements/Brick Solid  BrickDimensions=[4.5 0.7 8.6]  BrickDimensionsUnits=cm  ExportEntireGeometry=off  InertiaType=CalculateFromGeometry  BasedOnType=Density  Density=1000  DensityUnits=kg/m^3  Mass=1  MassUnits=kg  CenterOfMass=[0 0 0]  CenterOfMassUnits=m  MomentsOfInertia=[1 1 1]  MomentsOfInertiaUnits=kg*m^2  ProductsOfInertia=[0 0 0]  ProductsOfInertiaUnits=kg*m^2  GraphicType=FromGeometry  MarkerShape=Sphere  MarkerSize=10  GraphicVisPropType=SimpleVisualProperties  GraphicDiffuseColor=[0.5 0.5 0.5]  GraphicOpacity=1  GraphicSpecularColor=[0.5 0.5 0.5 1.0]  GraphicAmbientColor=[0.15 0.15 0.15 1.0]  GraphicEmissiveColor=[0.0 0.0 0.0 1.0]  GraphicShininess=75  DoExposeReferenceFrame=on  SerializedFrames=<Frames><Frame><Id>Frame1</Id><Value><Name>F1</Name><Origin><Source>ReferenceFrame</Source><FeatureName></FeatureName></Origin><PrimaryAxis><DefinedDirection>+Z</DefinedDirection><Source>ReferenceFrame</Source><SourceDirection>+Z</SourceDirection><FeatureName></FeatureName></PrimaryAxis><SecondaryAxis><DefinedDirection>+X</DefinedDirection><Source>ReferenceFrame</Source><SourceDirection>+X</SourceDirection><FeatureName></FeatureName></SecondaryAxis></Value></Frame></Frames>
  Brick Solid2 : sm_lib/Body Elements/Brick Solid  BrickDimensions=[4.5 0.7 8.6]  BrickDimensionsUnits=cm  ExportEntireGeometry=off  InertiaType=CalculateFromGeometry  BasedOnType=Density  Density=1000  DensityUnits=kg/m^3  Mass=1  MassUnits=kg  CenterOfMass=[0 0 0]  CenterOfMassUnits=m  MomentsOfInertia=[1 1 1]  MomentsOfInertiaUnits=kg*m^2  ProductsOfInertia=[0 0 0]  ProductsOfInertiaUnits=kg*m^2  GraphicType=FromGeometry  MarkerShape=Sphere  MarkerSize=10  GraphicVisPropType=SimpleVisualProperties  GraphicDiffuseColor=[0.5 0.5 0.5]  GraphicOpacity=1  GraphicSpecularColor=[0.5 0.5 0.5 1.0]  GraphicAmbientColor=[0.15 0.15 0.15 1.0]  GraphicEmissiveColor=[0.0 0.0 0.0 1.0]  GraphicShininess=75  DoExposeReferenceFrame=on  SerializedFrames=<Frames><Frame><Id>Frame1</Id><Value><Name>F1</Name><Origin><Source>ReferenceFrame</Source><FeatureName></FeatureName></Origin><PrimaryAxis><DefinedDirection>+Z</DefinedDirection><Source>ReferenceFrame</Source><SourceDirection>+Z</SourceDirection><FeatureName></FeatureName></PrimaryAxis><SecondaryAxis><DefinedDirection>+X</DefinedDirection><Source>ReferenceFrame</Source><SourceDirection>+X</SourceDirection><FeatureName></FeatureName></SecondaryAxis></Value></Frame></Frames>
  Flexible Angle Beam : sm_lib/Body Elements/Flexible Bodies/Beams/Flexible Angle Beam  EndToEndWidth=1  EndToEndWidthUnits=m  EndToEndHeight=1  EndToEndHeightUnits=m  VerticalLegThickness=0.1  VerticalLegThicknessUnits=m  HorizontalLegThickness=0.1  HorizontalLegThicknessUnits=m  Length=10  LengthUnits=m  StiffnessAndInertiaType=CalculateFromGeometry  Density=2700  DensityUnits=kg/m^3  ModuliType=YoungsPoissons  YoungsModulus=70  YoungsModulusUnits=GPa  PoissonsRatio=0.33  ShearModulus=26  ShearModulusUnits=GPa  GeometricCentroid=[0 0]  GeometricCentroidUnits=m  BendingCentroid=[0 0]  BendingCentroidUnits=m  ShearCenter=[0 0]  ShearCenterUnits=m  AxialRigidity=1  AxialRigidityUnits=Pa*m^2  FlexuralRigidity=[1 1]  FlexuralRigidityUnits=Pa*m^4  CrossFlexuralRigidity=0  CrossFlexuralRigidityUnits=Pa*m^4  TorsionalRigidity=1  TorsionalRigidityUnits=Pa*m^4  CenterOfMass=[0 0]  CenterOfMassUnits=m  MassPerUnitLength=1  MassPerUnitLengthUnits=kg/m  MassMomentOfInertiaDensity=[1 1]  MassMomentOfInertiaDensityUnits=kg*m  MassProductOfInertiaDensity=0  MassProductOfInertiaDensityUnits=kg*m  DampingType=Proportional  ProportionalDampingAlpha=0  ProportionalDampingAlphaUnits=1/s  ProportionalDampingBeta=0.001  ProportionalDampingBetaUnits=s  UniformModalDampingRatio=0.01  NumElements=1  ReferenceConditionsType=LinearizedMeanAxes  DoExposeReferenceFrame=off  ReductionType=None  NumRetainedModes=1  GraphicType=FromGeometry  GraphicVisPropType=SimpleVisualProperties  GraphicDiffuseColor=[0.5 0.5 0.5]  GraphicOpacity=1  GraphicSpecularColor=[0.5 0.5 0.5 1.0]  GraphicAmbientColor=[0.15 0.15 0.15 1.0]  GraphicEmissiveColor=[0.0 0.0 0.0 1.0]  GraphicShininess=75  DoExposeZminFrame=on  DoExposeZmaxFrame=on  SerializedFrames=<Frames/>
  Flexible Angle Beam1 : sm_lib/Body Elements/Flexible Bodies/Beams/Flexible Angle Beam  EndToEndWidth=1  EndToEndWidthUnits=m  EndToEndHeight=1  EndToEndHeightUnits=m  VerticalLegThickness=0.1  VerticalLegThicknessUnits=m  HorizontalLegThickness=0.1  HorizontalLegThicknessUnits=m  Length=10  LengthUnits=m  StiffnessAndInertiaType=CalculateFromGeometry  Density=2700  DensityUnits=kg/m^3  ModuliType=YoungsPoissons  YoungsModulus=70  YoungsModulusUnits=GPa  PoissonsRatio=0.33  ShearModulus=26  ShearModulusUnits=GPa  GeometricCentroid=[0 0]  GeometricCentroidUnits=m  BendingCentroid=[0 0]  BendingCentroidUnits=m  ShearCenter=[0 0]  ShearCenterUnits=m  AxialRigidity=1  AxialRigidityUnits=Pa*m^2  FlexuralRigidity=[1 1]  FlexuralRigidityUnits=Pa*m^4  CrossFlexuralRigidity=0  CrossFlexuralRigidityUnits=Pa*m^4  TorsionalRigidity=1  TorsionalRigidityUnits=Pa*m^4  CenterOfMass=[0 0]  CenterOfMassUnits=m  MassPerUnitLength=1  MassPerUnitLengthUnits=kg/m  MassMomentOfInertiaDensity=[1 1]  MassMomentOfInertiaDensityUnits=kg*m  MassProductOfInertiaDensity=0  MassProductOfInertiaDensityUnits=kg*m  DampingType=Proportional  ProportionalDampingAlpha=0  ProportionalDampingAlphaUnits=1/s  ProportionalDampingBeta=0.001  ProportionalDampingBetaUnits=s  UniformModalDampingRatio=0.01  NumElements=1  ReferenceConditionsType=LinearizedMeanAxes  DoExposeReferenceFrame=off  ReductionType=None  NumRetainedModes=1  GraphicType=FromGeometry  GraphicVisPropType=SimpleVisualProperties  GraphicDiffuseColor=[0.5 0.5 0.5]  GraphicOpacity=1  GraphicSpecularColor=[0.5 0.5 0.5 1.0]  GraphicAmbientColor=[0.15 0.15 0.15 1.0]  GraphicEmissiveColor=[0.0 0.0 0.0 1.0]  GraphicShininess=75  DoExposeZminFrame=on  DoExposeZmaxFrame=on  SerializedFrames=<Frames/>
  Flexible Angle Beam2 : sm_lib/Body Elements/Flexible Bodies/Beams/Flexible Angle Beam  EndToEndWidth=1  EndToEndWidthUnits=m  EndToEndHeight=1  EndToEndHeightUnits=m  VerticalLegThickness=0.1  VerticalLegThicknessUnits=m  HorizontalLegThickness=0.1  HorizontalLegThicknessUnits=m  Length=10  LengthUnits=m  StiffnessAndInertiaType=CalculateFromGeometry  Density=2700  DensityUnits=kg/m^3  ModuliType=YoungsPoissons  YoungsModulus=70  YoungsModulusUnits=GPa  PoissonsRatio=0.33  ShearModulus=26  ShearModulusUnits=GPa  GeometricCentroid=[0 0]  GeometricCentroidUnits=m  BendingCentroid=[0 0]  BendingCentroidUnits=m  ShearCenter=[0 0]  ShearCenterUnits=m  AxialRigidity=1  AxialRigidityUnits=Pa*m^2  FlexuralRigidity=[1 1]  FlexuralRigidityUnits=Pa*m^4  CrossFlexuralRigidity=0  CrossFlexuralRigidityUnits=Pa*m^4  TorsionalRigidity=1  TorsionalRigidityUnits=Pa*m^4  CenterOfMass=[0 0]  CenterOfMassUnits=m  MassPerUnitLength=1  MassPerUnitLengthUnits=kg/m  MassMomentOfInertiaDensity=[1 1]  MassMomentOfInertiaDensityUnits=kg*m  MassProductOfInertiaDensity=0  MassProductOfInertiaDensityUnits=kg*m  DampingType=Proportional  ProportionalDampingAlpha=0  ProportionalDampingAlphaUnits=1/s  ProportionalDampingBeta=0.001  ProportionalDampingBetaUnits=s  UniformModalDampingRatio=0.01  NumElements=1  ReferenceConditionsType=LinearizedMeanAxes  DoExposeReferenceFrame=off  ReductionType=None  NumRetainedModes=1  GraphicType=FromGeometry  GraphicVisPropType=SimpleVisualProperties  GraphicDiffuseColor=[0.5 0.5 0.5]  GraphicOpacity=1  GraphicSpecularColor=[0.5 0.5 0.5 1.0]  GraphicAmbientColor=[0.15 0.15 0.15 1.0]  GraphicEmissiveColor=[0.0 0.0 0.0 1.0]  GraphicShininess=75  DoExposeZminFrame=on  DoExposeZmaxFrame=on  SerializedFrames=<Frames/>
  Conn1 : PMIOPort  Side=Right
  Conn2 : PMIOPort  Port=2  Side=Left
  connections:
  Flexible Angle Beam/RConn1 -- Brick Solid1/LConn1
  Flexible Angle Beam2/LConn1 -- Brick Solid2/RConn1
  Flexible Angle Beam1/LConn1 -- Brick Solid1/RConn1
  Conn1/RConn1 -- Flexible Angle Beam/LConn1
  Flexible Angle Beam1/RConn1 -- Brick Solid2/LConn1
  Conn2/RConn1 -- Flexible Angle Beam2/RConn1

== matlab function soft_robot_model/MATLAB Function ==
  data: theta_x input; beta1 output; theta_y input; d_z input; L input; phi input; beta2 output; beta3 output
function [beta1, beta2, beta3] = kinematics(theta_x, theta_y, d_z, L, phi)
    % Base bending from height
    beta_base = 2 * acos(1 - d_z / (2*L));
    
    % Tilt projection onto each leg
    beta_tilt = theta_x * cos(phi) + theta_y * sin(phi);
    
    % Total bending per leg
    betas = beta_base + beta_tilt;
    
    beta1 = betas(1);
    beta2 = betas(2);
    beta3 = betas(3);
end
